simulink model "t_type_q1q4_switching_demo"  (R2025b)
settings: Solver=ode23t  StartTime=0.0  StopTime=t_stop_sw  MaxStep=max_step_sw  RelTol=1e-3
PreLoadFcn:
  | demo_root=fileparts(fileparts(get_param(bdroot,'FileName'))); run(fullfile(demo_root,'parameters','switching_demo_parameters.m')); clear demo_root;
undefined symbols (not defined in the file): m_index, Rd_sw, T_switch, Vdc_sw, w_grid_sw
libraries: ee_lib x11, nesl_utility x8, fl_lib x4, simulink x1
settings Model: Creator=bob  LastModifiedBy=bob

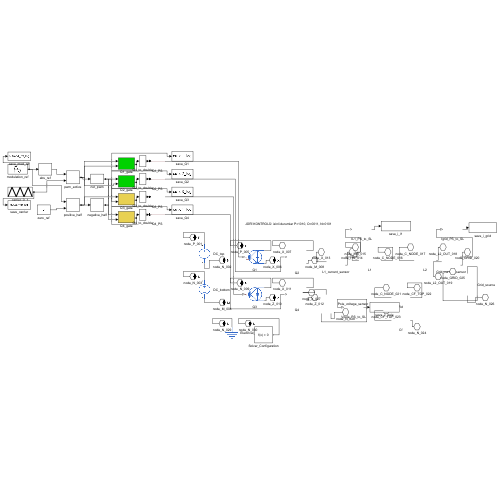
[thumbnail: Simulink's stored preview of the top-level diagram]
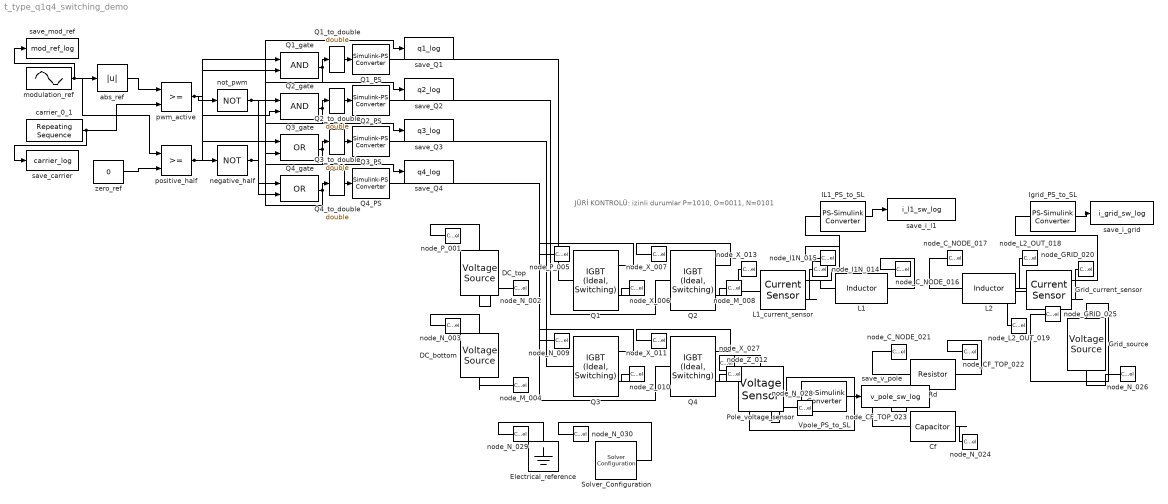
== system t_type_q1q4_switching_demo ==
  note: JÜRİ KONTROLÜ: izinli durumlar P=1010, O=0011, N=0101
  Cf : ee_lib/Passive/Capacitor  cap_option=ee.enum.passive.capacitor.capOption.const  c=Cf_sw F  Cvec=[1e-05, 1e-06] F  Vvec=[0, 10] V  CV_table_symmetry=ee.enum.passive.capacitor.tableSymmetry.yes  f_vec=[1, 10] kHz  DFext_vec=[.8, 1.2]  enable_C_tol=ee.enum.toleranceApplication.none  averaging_period=0 s  C_tol=5  tol_distribution=ee.enum.toleranceDistribution.uniform  nSigma=4  r=0 Ohm  g=0 1/Ohm  enable_operating_limits=ee.enum.enable.no  operating_limit_action=ee.enum.passive.reportOpLim.warn  max_working_voltage_range=[-25, 25] V  power_rating=1 W  maxTemperature=85 degC  thermalEnable=false  thermalMass=1 J/K  i_specify=off  i_priority=None  i=0 A  i_nominal_specify=off  i_nominal_value=1  i_nominal_unit=A  v_specify=off  v_priority=None  v=0 V  v_nominal_specify=off  v_nominal_value=1  v_nominal_unit=V  vc_specify=off  vc_priority=High  vc=0 V  vc_nominal_specify=off  vc_nominal_value=1  vc_nominal_unit=V  T_specify=off  T_priority=None  T=298.15 K  T_nominal_specify=off  T_nominal_value=1  T_nominal_unit=K
  DC_bottom : ee_lib/Sources/Voltage Source  dc_voltage=Vdc_sw/2 V  ac_voltage=0 V  ac_shift=0 rad  ac_frequency=60 Hz  noise_mode=ee.enum.sources.noise.Disabled  PSD=0 V^2/Hz  sample_time=1e-3 s  repeatability=ee.enum.sources.repeatability.NotRepeatable  user_seed=0  auto_seed=3890346746  i_specify=off  i_priority=None  i=0 A  i_nominal_specify=off  i_nominal_value=1  i_nominal_unit=A  v_specify=off  v_priority=None  v=0 V  v_nominal_specify=off  v_nominal_value=1  v_nominal_unit=V
  DC_top : ee_lib/Sources/Voltage Source  dc_voltage=Vdc_sw/2 V  ac_voltage=0 V  ac_shift=0 rad  ac_frequency=60 Hz  noise_mode=ee.enum.sources.noise.Disabled  PSD=0 V^2/Hz  sample_time=1e-3 s  repeatability=ee.enum.sources.repeatability.NotRepeatable  user_seed=0  auto_seed=3499211588  i_specify=off  i_priority=None  i=0 A  i_nominal_specify=off  i_nominal_value=1  i_nominal_unit=A  v_specify=off  v_priority=None  v=0 V  v_nominal_specify=off  v_nominal_value=1  v_nominal_unit=V
  Electrical_reference : fl_lib/Electrical/Electrical Elements/Electrical Reference
  Grid_current_sensor : fl_lib/Electrical/Electrical Sensors/Current Sensor
  Grid_source : ee_lib/Sources/Voltage Source  dc_voltage=0 V  ac_voltage=V_grid_pk_sw V  ac_shift=0 rad  ac_frequency=f_grid_sw Hz  noise_mode=ee.enum.sources.noise.Disabled  PSD=0 V^2/Hz  sample_time=1e-3 s  repeatability=ee.enum.sources.repeatability.NotRepeatable  user_seed=0  auto_seed=545404223  i_specify=off  i_priority=None  i=0 A  i_nominal_specify=off  i_nominal_value=1  i_nominal_unit=A  v_specify=off  v_priority=None  v=0 V  v_nominal_specify=off  v_nominal_value=1  v_nominal_unit=V
  IL1_PS_to_SL : nesl_utility/PS-Simulink Converter  PhysicalDomain=network_engine_domain  SubClassName=ps_output  LeftPortType=input  RightPortType=output  PseudoPeriodic=off  Frequencies=[]  VectorFormat=inherit  Unit=A  AffineConversion=off
  Igrid_PS_to_SL : nesl_utility/PS-Simulink Converter  PhysicalDomain=network_engine_domain  SubClassName=ps_output  LeftPortType=input  RightPortType=output  PseudoPeriodic=off  Frequencies=[]  VectorFormat=inherit  Unit=A  AffineConversion=off
  L1 : ee_lib/Passive/Inductor  l=L1_sw H  enable_L_tol=ee.enum.toleranceApplication.none  L_tol=20  tol_distribution=ee.enum.toleranceDistribution.uniform  nSigma=4  r=R1_sw Ohm  g=1e-9 1/Ohm  enable_operating_limits=ee.enum.enable.no  operating_limit_action=ee.enum.passive.reportOpLim.warn  max_working_current=1 A  power_rating=1 W  i_L_specify=off  i_L_priority=High  i_L=0 A  i_L_nominal_specify=off  i_L_nominal_value=1  i_L_nominal_unit=A
  L1_current_sensor : fl_lib/Electrical/Electrical Sensors/Current Sensor
  L2 : ee_lib/Passive/Inductor  l=L2_sw H  enable_L_tol=ee.enum.toleranceApplication.none  L_tol=20  tol_distribution=ee.enum.toleranceDistribution.uniform  nSigma=4  r=R2_sw Ohm  g=1e-9 1/Ohm  enable_operating_limits=ee.enum.enable.no  operating_limit_action=ee.enum.passive.reportOpLim.warn  max_working_current=1 A  power_rating=1 W  i_L_specify=off  i_L_priority=High  i_L=0 A  i_L_nominal_specify=off  i_L_nominal_value=1  i_L_nominal_unit=A
  Pole_voltage_sensor : fl_lib/Electrical/Electrical Sensors/Voltage Sensor
  Q{1..4} (4 alike) : ee_lib/Semiconductors & Converters/IGBT (Ideal, Switching)  port_option=ee.enum.controlport.ps  Vf=Vf_sw V  Ron=Ron_sw Ohm  Goff=Goff_sw 1/Ohm  Vth=Vth_sw V  diode_param=ee.enum.semiconductors.protectionDiode.nodynamics  diode_Vf=0.8 V  diode_Ron=0.001 Ohm  diode_Goff=1e-5 1/Ohm  diode_C=50e-9 F  diode_iRM=-235 A  diode_iF=300 A  diode_idot=-50 A/us  diode_trr_param=ee.enum.converters.diodeReverseParam.trr_factor  diode_trr_factor=3  diode_trr=15 us  diode_Qrr=1500 s*uA  ice_specify=off  ice_priority=None  ice=0 A  ice_nominal_specify=off  ice_nominal_value=1  ice_nominal_unit=A  vce_specify=off  vce_priority=None  vce=0 V  vce_nominal_specify=off  vce_nominal_value=1  vce_nominal_unit=V  vge_specify=off  vge_priority=None  vge=0 V  vge_nominal_specify=off  vge_nominal_value=1  vge_nominal_unit=V  thermal_loss_option=ee.enum.converters.thermalLossOption.constantvalues  Von_data=[0, .1, .6, .8, 1, 1.3, 1.6, 2, 2.4; 0, .1, .7, 1, 1.2, 1.5, 1.9, 2.4, 2.8] V  Tj=[298.15, 398.15] K  Iout_data=[0, .1, 1, 5, 10, 20, 40, 70, 100] A  Eon_data=[0, .0024, .024, .12, .2, .48, 1.04, 2.16, 3.24; 0, .003, .03, .15, .25, .6, 1.3, 2.7, 4.05] * 1e-3 J  Eoff_data=[0, .0007, .0066, .033, .066, .17, .33, .83, 1.5; 0, .001, .01, .05, .1, .25, .5, 1.2, 2.2] * 1e-3 J  Eon_data_3D=[zeros(2, 9, 3)] J  Eoff_data_3D=[zeros(2, 9, 3)] J  Tj_loss=[298.15, 398.15] K  Iout_data_loss=[0, .1, 1, 5, 10, 20, 40, 70, 100] A  tabulateWithVce=false  Vce_loss=[0, 150, 300] V  Eon_scalar=22.86e-3 J  Eoff_scalar=17.14e-3 J  Voff=300 V  Iout_scalar=600 A  useCurrentFromPreviousCycle=false  useVoltageFromPreviousCycle=false  diodeModelType=ee.enum.converters.diodeModelType.pwl  diodeTableType=ee.enum.diode.tableType.IfMat  diode_ReverseIVType=ee.enum.diode.diodeReverseIV.constant  diode_IfMat=[.07, .12, .19, 1.75, 4.24, 7.32, 11.2; .16, .3, .72, 2.14, 4.02, 6.35, 9.12] A  diode_VfMat=[.9, 1.15, 1.25, 1.5, 1.75, 2.17, 2.6, 2.85; .58, .68, .75, 1.1, 1.38, 1.77, 2.27, 2.7] V  diode_TjVec=[25, 125] degC  diode_VfVec=[.5, .7, .9, 1.3, 1.7, 2.1, 2.5] V  diode_IfVec=[.1, .2, .5, 1, 2, 4, 7, 10] A  diode_IrMat=[1e-06, 2e-06, 5e-06, 1e-05, 2.5e-05, 5e-05, .0001; 2e-06, 5e-06, 1e-05, 4e-05, 8e-05, .0002, .0005] A  diode_VrMat=[10, 100, 200, 250, 300, 325, 350; 10, 70, 160, 220, 270, 300, 320] V  diode_VrVec=[10, 20, 40, 50, 70, 80, 100] V  diode_IrVec=[1e-06, 2e-06, 5e-06, 1e-05, 2e-05, 5e-05, .0001] A  diode_Vr=-600 V  diode_Ls=150 nH  diode_Erec=0.03 J  diode_rec_loss_model=ee.enum.diode.reverseRecoveryModel.fixed  diode_ErecVal=0 J  diode_scaleWithIandV=true  diode_ErecMat=zeros(2, 3) J  diode_TjrecVec=[298.15, 398.15] K  diode_IfrecVec=[.1, 1, 10] A  diode_IrecVal=10 A  diode_VrecVal=10 V  diode_tFilter=1 / 1000 / 100 s  separateThermalPortForDiode=false  thermal_network_parameterization=ee.enum.thermalNetworkTopology.external  Rth=[.08, .5] K/W  Rth_Cauer=[.08, .1, .5] K/W  Rth_Foster=[.08, .14, .22, .16] K/W  thermal_mass_parameterization=ee.enum.thermalNetwork.timeconstant  thermal_mass=[.01, .5] J/K  thermal_mass_Cauer=[.01, .1, .5] J/K  thermal_mass_Foster=[.001, .005, .05, .5] J/K  thermal_time_constant=[.001, .2] s  thermal_time_constant_Cauer=[.001, .1, .2] s  thermal_time_constant_Foster=[7e-05, .0007, .01, .08] s  thermal_mass_initial_temperatures=[25, 25] degC  thermal_mass_initial_temperatures_Cauer=[25, 25, 25] degC  junction_thermal_mass=0.01 J/K  Tvec_initial_Foster=[25, 25, 25, 25] degC  RthDiode=[.03, .2] K/W  RthCauerDiode=[.03, .1, .2] K/W  RthFosterDiode=[.03, .2] K/W  thermalMassDiode=[3, 25] J/K  thermalMassCauerDiode=[3, 10, 25] J/K  thermalMassFosterDiode=[33, 50] J/K  thermalTauDiode=[.1, 5] s  thermalTauCauerDiode=[.1, 1, 5] s  thermalTauFosterDiode=[1, 10] s  thermalMassInitTempDiode=[25, 25] degC  thermalMassInitTempCauerDiode=[25, 25, 25] degC  junctionthermalMassDiode=0.1 J/K  TVecInitialFosterDiode=[25, 25, 25, 25] degC  no_thermal_network=0  IGBT_junction_temperature_specify=off  IGBT_junction_temperature_priority=None  IGBT_junction_temperature=25 degC  IGBT_junction_temperature_nominal_specify=off  IGBT_junction_temperature_nominal_value=1  IGBT_junction_temperature_nominal_unit=degC  diode_junction_temperature_specify=off  diode_junction_temperature_priority=None  diode_junction_temperature=25 degC  diode_junction_temperature_nominal_specify=off  diode_junction_temperature_nominal_value=1  diode_junction_temperature_nominal_unit=degC  Qj_specify=off  Qj_priority=None  Qj=0 W  Qj_nominal_specify=off  Qj_nominal_value=1  Qj_nominal_unit=W  accumulatedSwitchingLosses_specify=off  accumulatedSwitchingLosses_priority=None  accumulatedSwitchingLosses=0 J
  Q1_PS : nesl_utility/Simulink-PS Converter  PhysicalDomain=network_engine_domain  SubClassName=ps_input  LeftPortType=input  RightPortType=output  PseudoPeriodic=off  Frequencies=[]  NoiseDistribution=none  NoiseParameters=[]  Unit=V  AffineConversion=off  FilteringAndDerivatives=zero  SimscapeFilterOrder=1  InputFilterTimeConstant=0.001  UdotUserProvided=0
  Q1_gate : Logic  AllPortsSameDT=off  OutDataTypeStr=boolean
  Q1_to_double : DataTypeConversion  OutDataTypeStr=double  SaturateOnIntegerOverflow=off  RndMeth=Floor
  Q2_PS : nesl_utility/Simulink-PS Converter  PhysicalDomain=network_engine_domain  SubClassName=ps_input  LeftPortType=input  RightPortType=output  PseudoPeriodic=off  Frequencies=[]  NoiseDistribution=none  NoiseParameters=[]  Unit=V  AffineConversion=off  FilteringAndDerivatives=zero  SimscapeFilterOrder=1  InputFilterTimeConstant=0.001  UdotUserProvided=0
  Q2_gate : Logic  AllPortsSameDT=off  OutDataTypeStr=boolean
  Q2_to_double : DataTypeConversion  OutDataTypeStr=double  SaturateOnIntegerOverflow=off  RndMeth=Floor
  Q3_PS : nesl_utility/Simulink-PS Converter  PhysicalDomain=network_engine_domain  SubClassName=ps_input  LeftPortType=input  RightPortType=output  PseudoPeriodic=off  Frequencies=[]  NoiseDistribution=none  NoiseParameters=[]  Unit=V  AffineConversion=off  FilteringAndDerivatives=zero  SimscapeFilterOrder=1  InputFilterTimeConstant=0.001  UdotUserProvided=0
  Q3_gate : Logic  Operator=OR  AllPortsSameDT=off  OutDataTypeStr=boolean
  Q3_to_double : DataTypeConversion  OutDataTypeStr=double  SaturateOnIntegerOverflow=off  RndMeth=Floor
  Q4_PS : nesl_utility/Simulink-PS Converter  PhysicalDomain=network_engine_domain  SubClassName=ps_input  LeftPortType=input  RightPortType=output  PseudoPeriodic=off  Frequencies=[]  NoiseDistribution=none  NoiseParameters=[]  Unit=V  AffineConversion=off  FilteringAndDerivatives=zero  SimscapeFilterOrder=1  InputFilterTimeConstant=0.001  UdotUserProvided=0
  Q4_gate : Logic  Operator=OR  AllPortsSameDT=off  OutDataTypeStr=boolean
  Q4_to_double : DataTypeConversion  OutDataTypeStr=double  SaturateOnIntegerOverflow=off  RndMeth=Floor
  Rd : ee_lib/Passive/Resistor  R=Rd_sw Ohm  enable_R_tol=ee.enum.toleranceApplication.none  R_tol=5  tol_distribution=ee.enum.toleranceDistribution.uniform  nSigma=4  enable_operating_limits=ee.enum.enable.no  operating_limit_action=ee.enum.passive.reportOpLim.warn  power_rating=1 W  max_working_voltage=100 V  noise_mode=ee.enum.sources.noise.Disabled  Tdevice=25 degC  sample_time=1e-3 s  repeatability=ee.enum.ic.repeatability.notRepeatable  user_seed=0  auto_seed=3922919431  power_derating_T1=70 degC  power_derating_T2=155 degC  operating_temperature_range_vec=[-50, 150] degC  alpha=3.93e-3 1/K  Tmeas=25 degC  thermal_mass=100 J/K  temperature_specify=off  temperature_priority=High  temperature=298.15 K  temperature_nominal_specify=off  temperature_nominal_value=1  temperature_nominal_unit=K
  Solver_Configuration : nesl_utility/Solver Configuration  PhysicalDomain=network_engine_domain  SubClassName=solver  LeftPortType=input  RightPortType=generic  Tones=[]  Harmonics=[]  SimulateNoise=off  Profile=off  UseLocalSampling=off  EnableSwitchedLinearOptims=on  FrequencyDomain=off  UseCCode=off  RelTol=0.001  AbsTol=0.001  MinStep=1e-09  ToWorkspace=off  RevertToSquareIcSolve=off  NumHomotopyIterations=100  PhasorMode=off  PhasorModeNumHarmonics=1  ConsistencySolver=NEWTON_XTOL_AFTER_FTOL  IndexReductionMethod=DerivativeReplacement  DoDC=off  ResidualTolerance=1e-09  ConsistencyTolSource=GLOBAL  ConsistencyAbsTol=0.001  ConsistencyRelTol=0.001  ConsistencyTolFactor=0.001  UseLocalSolver=off  LocalSolverChoice=NE_BACKWARD_EULER_ADVANCER  ResolveIndetEquations=on  FunctionEvalNumThread=1  LocalSolverSampleTime=0.001  DoFixedCost=off  MaxNonlinIter=3  MaxModeIter=2  ComputeImpulses=off  ImpulseIterations=2  LinearAlgebra=auto  LinearAlgebraNumThread=0  EquationFormulation=NE_TIME_EF  DelaysMemoryBudget=1024  AutomaticFiltering=on  FilteringTimeConstant=0.001  PartitionStorageMethod=AS_NEEDED  PartitionMemoryBudget=1024  PartitionMethod=ROBUST  MultibodyUseLocalSolver=off  MultibodyLocalSolverChoice=ODE1  MultibodyLocalSolverSampleTime=0.001
  Vpole_PS_to_SL : nesl_utility/PS-Simulink Converter  PhysicalDomain=network_engine_domain  SubClassName=ps_output  LeftPortType=input  RightPortType=output  PseudoPeriodic=off  Frequencies=[]  VectorFormat=inherit  Unit=V  AffineConversion=off
  abs_ref : Abs  SaturateOnIntegerOverflow=off
  carrier_0_1 : simulink/Sources/Repeating Sequence  rep_seq_t=[0 T_switch/2 T_switch]  rep_seq_y=[0 1 0]
  modulation_ref : Sin  Amplitude=m_index  Frequency=w_grid_sw  SampleTime=0
  negative_half : Logic  Operator=NOT  AllPortsSameDT=off  OutDataTypeStr=boolean
  node_CF_TOP_022 : ConnectionLabel  Label=CF_TOP
  node_CF_TOP_023 : ConnectionLabel  Label=CF_TOP
  node_C_NODE_016 : ConnectionLabel  Label=C_NODE
  node_C_NODE_017 : ConnectionLabel  Label=C_NODE
  node_C_NODE_021 : ConnectionLabel  Label=C_NODE
  node_GRID_020 : ConnectionLabel  Label=GRID
  node_GRID_025 : ConnectionLabel  Label=GRID
  node_I1N_014 : ConnectionLabel  Label=I1N
  node_I1N_015 : ConnectionLabel  Label=I1N
  node_L2_OUT_018 : ConnectionLabel  Label=L2_OUT
  node_L2_OUT_019 : ConnectionLabel  Label=L2_OUT
  node_M_004 : ConnectionLabel  Label=M
  node_M_008 : ConnectionLabel  Label=M
  node_N_002 : ConnectionLabel  Label=N
  node_N_003 : ConnectionLabel  Label=N
  node_N_009 : ConnectionLabel  Label=N
  node_N_024 : ConnectionLabel  Label=N
  node_N_026 : ConnectionLabel  Label=N
  node_N_028 : ConnectionLabel  Label=N
  node_N_029 : ConnectionLabel  Label=N
  node_N_030 : ConnectionLabel  Label=N
  node_P_001 : ConnectionLabel  Label=P
  node_P_005 : ConnectionLabel  Label=P
  node_X_006 : ConnectionLabel  Label=X
  node_X_007 : ConnectionLabel  Label=X
  node_X_011 : ConnectionLabel  Label=X
  node_X_013 : ConnectionLabel  Label=X
  node_X_027 : ConnectionLabel  Label=X
  node_Z_010 : ConnectionLabel  Label=Z
  node_Z_012 : ConnectionLabel  Label=Z
  not_pwm : Logic  Operator=NOT  AllPortsSameDT=off  OutDataTypeStr=boolean
  positive_half : RelationalOperator  OutDataTypeStr=boolean  RndMeth=Simplest  InputSameDT=off
  pwm_active : RelationalOperator  OutDataTypeStr=boolean  RndMeth=Simplest  InputSameDT=off
  save_Q1 : ToWorkspace  VariableName=q1_log  SaveFormat=Timeseries  SampleTime=-1
  save_Q2 : ToWorkspace  VariableName=q2_log  SaveFormat=Timeseries  SampleTime=-1
  save_Q3 : ToWorkspace  VariableName=q3_log  SaveFormat=Timeseries  SampleTime=-1
  save_Q4 : ToWorkspace  VariableName=q4_log  SaveFormat=Timeseries  SampleTime=-1
  save_carrier : ToWorkspace  VariableName=carrier_log  SaveFormat=Timeseries  SampleTime=-1
  save_i_grid : ToWorkspace  VariableName=i_grid_sw_log  SaveFormat=Timeseries  SampleTime=-1
  save_i_l1 : ToWorkspace  VariableName=i_l1_sw_log  SaveFormat=Timeseries  SampleTime=-1
  save_mod_ref : ToWorkspace  VariableName=mod_ref_log  SaveFormat=Timeseries  SampleTime=-1
  save_v_pole : ToWorkspace  VariableName=v_pole_sw_log  SaveFormat=Timeseries  SampleTime=-1
  zero_ref : Constant  Value=0
  wires:
  modulation_ref/1 -> abs_ref/1, positive_half/1, save_mod_ref/1
  abs_ref/1 -> pwm_active/1
  carrier_0_1/1 -> pwm_active/2, save_carrier/1
  zero_ref/1 -> positive_half/2
  positive_half/1 -> negative_half/1, Q1_gate/1, Q3_gate/1
  pwm_active/1 -> not_pwm/1, Q1_gate/2, Q2_gate/2
  negative_half/1 -> Q2_gate/1, Q4_gate/1
  not_pwm/1 -> Q3_gate/2, Q4_gate/2
  Q1_gate/1 -> Q1_to_double/1, save_Q1/1
  Q1_to_double/1 -> Q1_PS/1
  Q2_gate/1 -> Q2_to_double/1, save_Q2/1
  Q2_to_double/1 -> Q2_PS/1
  Q3_gate/1 -> Q3_to_double/1, save_Q3/1
  Q3_to_double/1 -> Q3_PS/1
  Q4_gate/1 -> Q4_to_double/1, save_Q4/1
  Q4_to_double/1 -> Q4_PS/1
  IL1_PS_to_SL/1 -> save_i_l1/1
  Igrid_PS_to_SL/1 -> save_i_grid/1
  Vpole_PS_to_SL/1 -> save_v_pole/1
  connections:
  Q1_PS/RConn1 -- Q1/LConn1
  Q2_PS/RConn1 -- Q2/LConn1
  Q3_PS/RConn1 -- Q3/LConn1
  Q4_PS/RConn1 -- Q4/LConn1
  DC_top/LConn1 -- node_P_001/LConn1
  DC_top/RConn1 -- node_N_002/LConn1
  DC_bottom/LConn1 -- node_N_003/LConn1
  DC_bottom/RConn1 -- node_M_004/LConn1
  Q1/RConn1 -- node_P_005/LConn1
  Q1/RConn2 -- node_X_006/LConn1
  Q2/RConn1 -- node_X_007/LConn1
  Q2/RConn2 -- node_M_008/LConn1
  Q3/RConn1 -- node_N_009/LConn1
  Q3/RConn2 -- node_Z_010/LConn1
  Q4/RConn1 -- node_X_011/LConn1
  Q4/RConn2 -- node_Z_012/LConn1
  L1_current_sensor/LConn1 -- node_X_013/LConn1
  L1_current_sensor/RConn2 -- node_I1N_014/LConn1
  L1/LConn1 -- node_I1N_015/LConn1
  L1/RConn1 -- node_C_NODE_016/LConn1
  L2/LConn1 -- node_C_NODE_017/LConn1
  L2/RConn1 -- node_L2_OUT_018/LConn1
  Grid_current_sensor/LConn1 -- node_L2_OUT_019/LConn1
  Grid_current_sensor/RConn2 -- node_GRID_020/LConn1
  Rd/LConn1 -- node_C_NODE_021/LConn1
  Rd/RConn1 -- node_CF_TOP_022/LConn1
  Cf/LConn1 -- node_CF_TOP_023/LConn1
  Cf/RConn1 -- node_N_024/LConn1
  Grid_source/LConn1 -- node_GRID_025/LConn1
  Grid_source/RConn1 -- node_N_026/LConn1
  Pole_voltage_sensor/LConn1 -- node_X_027/LConn1
  Pole_voltage_sensor/RConn2 -- node_N_028/LConn1
  Electrical_reference/LConn1 -- node_N_029/LConn1
  Solver_Configuration/RConn1 -- node_N_030/LConn1
  L1_current_sensor/RConn1 -- IL1_PS_to_SL/LConn1
  Grid_current_sensor/RConn1 -- Igrid_PS_to_SL/LConn1
  Pole_voltage_sensor/RConn1 -- Vpole_PS_to_SL/LConn1
